simulink model "PI_control"  (R2025b)
settings: Solver=VariableStepAuto  StartTime=0.0  StopTime=50  RelTol=1e-3
libraries: simulink x2, slpidlib x1
settings Model: Creator=feder  LastModifiedBy=feder

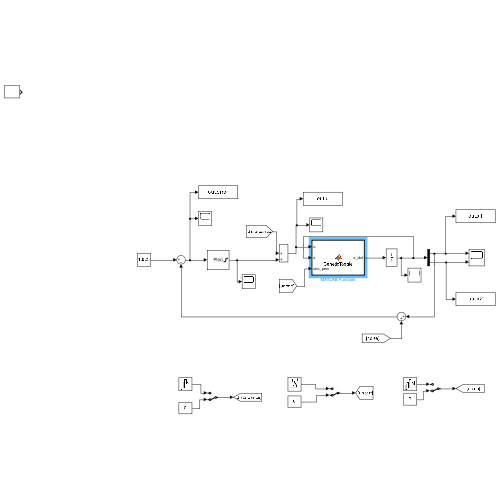
[thumbnail: Simulink's stored preview of the top-level diagram]
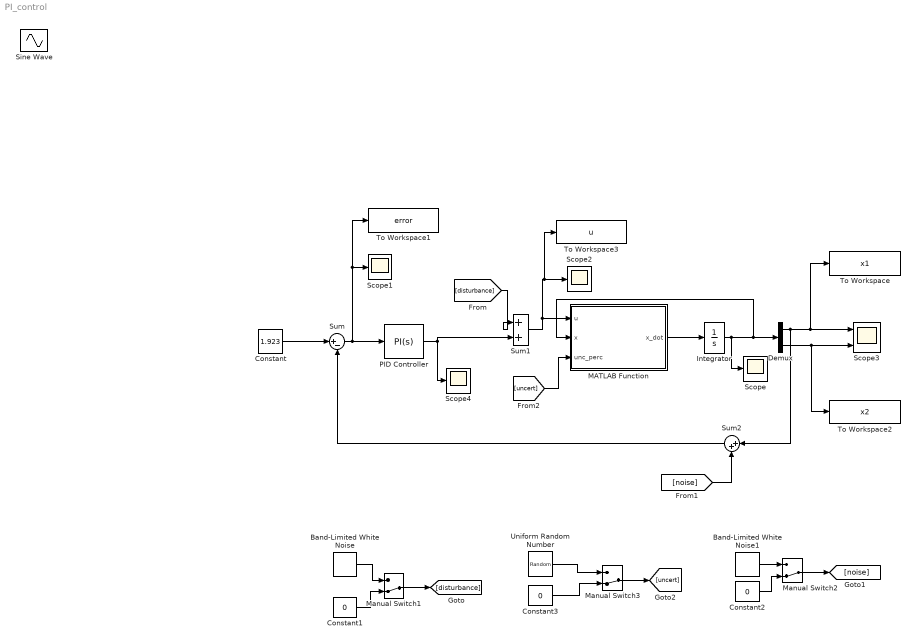
== system PI_control ==
  Band-Limited White Noise : simulink/Sources/Band-Limited White Noise  Cov=[0.001]  Ts=0.01  seed=[23341]
  Band-Limited White Noise1 : simulink/Sources/Band-Limited White Noise  Cov=[10]  Ts=0.1  seed=[23341]
  Constant : Constant  Value=1.923
  Constant1 : Constant  Value=0
  Constant2 : Constant  Value=0
  Constant3 : Constant  Value=0
  Demux : Demux  Outputs=2
  Integrator : Integrator  InitialCondition=[0.12;7.8]
  MATLAB Function : MATLAB Function  TreatAsAtomicUnit=on
  Manual Switch1 : ManualSwitch  CurrentSetting=0
  Manual Switch2 : ManualSwitch  CurrentSetting=0
  Manual Switch3 : ManualSwitch  CurrentSetting=0
  PID Controller : slpidlib/PID Controller  Controller=PI  Form=Parallel  TimeDomain=Continuous-time  UseExternalTs=off  SampleTime=-1  IntegratorMethod=Forward Euler  FilterMethod=Forward Euler  ControllerParametersSource=internal  P=1300  I=130000  UseKiTs=off  D=3000  UseExternalDerivativeSource=off  N=100  UseFilter=on  TunerSelectOption=Transfer Function Based (PID Tuner App)  InitialConditionSource=internal  InitialConditionForIntegrator=0  InitialConditionForFilter=0  DifferentiatorICPrevScaledInput=0  ExternalReset=none  TrackingMode=off  Kt=1  LimitOutput=on  SatLimitsSource=internal  UpperSaturationLimit=30  LowerSaturationLimit=-10  LinearizeAsGain=on  AntiWindupMode=none  Kb=1  LimitIntegrator=on  UpperIntegratorSaturationLimit=30  LowerIntegratorSaturationLimit=-10  POutMin=[]  POutMax=[]  IOutMin=[]  IOutMax=[]  DOutMin=[]  DOutMax=[]  NOutMin=[]  NOutMax=[]  SumOutMin=[]  SumOutMax=[]  SaturationOutMin=[]  SaturationOutMax=[]  PParamMin=[]  PParamMax=[]  IParamMin=[]  IParamMax=[]  DParamMin=[]  DParamMax=[]  NParamMin=[]  NParamMax=[]  KbParamMin=[]  KbParamMax=[]  KtParamMin=[]  KtParamMax=[]  KbOutMin=[]  KbOutMax=[]  KtOutMin=[]  KtOutMax=[]  IntegratorOutMin=[]  IntegratorOutMax=[]  FilterOutMin=[]  FilterOutMax=[]  SumI1OutMin=[]  SumI1OutMax=[]  SumI2OutMin=[]  SumI2OutMax=[]  SumI3OutMin=[]  SumI3OutMax=[]  SumI4OutMin=[]  SumI4OutMax=[]  SumDOutMin=[]  SumDOutMax=[]  DifferentiatorOutMin=[]  DifferentiatorOutMax=[]  FilterDiffOutCoefMin=[]  FilterDiffOutCoefMax=[]  ReciprocalOutMin=[]  ReciprocalOutMax=[]  SumDenOutMin=[]  SumDenOutMax=[]  SumNumOutMin=[]  SumNumOutMax=[]  DivideOutMin=[]  DivideOutMax=[]  UdiffTsProdOutMin=[]  UdiffTsProdOutMax=[]  NTsProdOutMin=[]  NTsProdOutMax=[]  UintegralTsProdOutMin=[]  UintegralTsProdOutMax=[]  UngainTsProdOutMin=[]  UngainTsProdOutMax=[]  ClampingZeroOutDataTypeStr=Inherit: Inherit via back propagation  ClampingZeroOutMin=[]  ClampingZeroOutMax=[]  FilterDenConstantOutDataTypeStr=Inherit: Inherit via back propagation  FilterDenConstantOutMin=[]  FilterDenConstantOutMax=[]  PCopyOutDataTypeStr=Inherit: Inherit via back propagation  PCopyOutMin=[]  PCopyOutMax=[]  NCopyOutDataTypeStr=Inherit: Inherit via back propagation  NCopyOutMin=[]  NCopyOutMax=[]  IntegratorContinuousStateAttributes=''  IntegratorStateMustResolveToSignalObject=off  IntegratorRTWStateStorageClass=Auto  FilterContinuousStateAttributes=''  FilterStateMustResolveToSignalObject=off  FilterRTWStateStorageClass=Auto  ParallelPVariant=InternalParameters  IdealPVariant=Disabled  IVariant=InternalParameters  DVariant=Disabled  IntegratorVariant=Continuous  SatVariant=Enabled  AWVariant=Passthrough  PCopyVariant=Disabled  TRVariant=Disabled  FdbkBlocksVariant=Forward  IdealPFdbkVariant=Disabled  SatFdbkVariant=Disabled  DerivativeFilterVariant=Disabled  NVariant=Disabled  NCopyVariant=Disabled_SignalSpec  FilterICVariant=Disabled  IntegratorICVariant=InternalICs  ExternalResetVariant=Disabled  TRSumVariant=Passthrough  SumFdbkVariant=Disabled  SumVariant=Sum_PI  TsampFilterVariant=InternalTs  TsampNgainVariant=Passthrough  TsampIntegralVariant=Disabled_SignalSpec  ExternalSaturationOutDataTypeStr=Inherit: Same as second input  DerivativeSourceVariant=Disabled  PreIntVariant=InternalPreInt
  Scope{,1..2,4} (4 alike) : Scope
      Scope settings: ActiveDisplayYMinimum=-9.8069508288691782  ActiveDisplayYMaximum=14.451771046736985
      Scope1 settings: ActiveDisplayYMinimum=-34.783607825873048  ActiveDisplayYMaximum=51.613721318170718
      Scope2 settings: ActiveDisplayYMinimum=-3.7469347766772851  ActiveDisplayYMaximum=33.74965941963081  DataLoggingVariableName=ScopeData2
      Scope4 settings: ActiveDisplayYMinimum=-3.7469347766774233  ActiveDisplayYMaximum=33.749659419630824  DataLoggingVariableName=ScopeData4
  Scope3 : Scope  NumInputPorts=2
      settings: ActiveDisplayYMinimum=-0.12809356838326824  ActiveDisplayYMaximum=2.1947048257052804  DataLoggingVariableName=ScopeData3
  Sine Wave : Sin  Amplitude=4  SampleTime=0
  Sum : Sum  Inputs=|+-
  Sum1 : Sum  Inputs=|++
  Sum2 : Sum  Inputs=|++
  To Workspace : ToWorkspace  VariableName=x1  SaveFormat=Timeseries  SampleTime=-1
  To Workspace1 : ToWorkspace  VariableName=error  SaveFormat=Timeseries  SampleTime=-1
  To Workspace2 : ToWorkspace  VariableName=x2  SaveFormat=Timeseries  SampleTime=-1
  To Workspace3 : ToWorkspace  VariableName=u  SaveFormat=Timeseries  SampleTime=-1
  Uniform Random Number : UniformRandomNumber  Minimum=-0.2  Maximum=0.2  SampleTime=5
  wires:
  MATLAB Function/1(x_dot) -> Integrator/1
  Integrator/1 -> Scope/1, MATLAB Function/2(x), Demux/1
  Demux/1 -> Sum2/1, To Workspace/1, Scope3/1
  Sum/1 -> To Workspace1/1, Scope1/1, PID Controller/1
  Constant1/1 -> Manual Switch1/2
  Manual Switch1/1 -> [disturbance]
  PID Controller/1 -> Scope4/1, Sum1/2
  [disturbance] -> Sum1/1
  Sum1/1 -> To Workspace3/1, Scope2/1, MATLAB Function/1(u)
  Demux/2 -> To Workspace2/1, Scope3/2
  Constant2/1 -> Manual Switch2/2
  Band-Limited White Noise1/1 -> Manual Switch2/1
  Manual Switch2/1 -> [noise]
  [noise] -> Sum2/2
  Sum2/1 -> Sum/2
  Uniform Random Number/1 -> Manual Switch3/1
  Constant3/1 -> Manual Switch3/2
  Manual Switch3/1 -> [uncert]
  [uncert] -> MATLAB Function/3(unc_perc)
  Constant/1 -> Sum/1
  Band-Limited White Noise/1 -> Manual Switch1/1

== matlab function PI_control/MATLAB Function ==
  data: u input; x_dot output; x input; unc_perc input
function x_dot = GeneticToggle(u, x, unc_perc)
 
    alpha_Y_nom = 10;   % Tasso di produzione nominale Proteina 1
    alpha_Z     = 10;   % Tasso di produzione nominale Proteina 2
  
    beta_Y  = 0.25;     % Parametri di resource sequestration
    beta_Z  = 0.25;
    
    gamma_Y = 1;        % Tassi di degradazione
    gamma_Z = 1;
    
    K_Y = 1; K_Z = 1;   % Costanti di dissociazione
    n = 2;              % Coefficiente di Hill (Cooperatività)

    x1 = x(1);
    x2 = x(2);


    % Il parametro alpha reale varia rispetto al nominale in base a unc_perc.

    alpha_Y_effettiva = alpha_Y_nom * (1 + unc_perc);
    alpha_Y_act = alpha_Y_effettiva + u;

    if alpha_Y_act < 0
        alpha_Y_act = 0;
    end

    % Hill_Z: Quanto x2 reprime x1
    Hill_Z = 1 / (1 + (x2/K_Z)^n);
    % Hill_Y: Quanto x1 reprime x2
    Hill_Y = 1 / (1 + (x1/K_Y)^n);

    %Denominatore
    % Più i geni sono attivi, più risorse (ribosomi) sequestrano.
    D = 1 + beta_Y * Hill_Z + beta_Z * Hill_Y;

    % Dinamica x1 (controllata)
    dx1 = (alpha_Y_act * Hill_Z / D) - gamma_Y * x1;
    
    % Dinamica x2 (non controllata direttamente)
    dx2 = (alpha_Z     * Hill_Y / D) - gamma_Z * x2;

    % Output
    x_dot = [dx1; dx2];
end
